simulink model "DCHR_Dispatch_Stateflow_v40"  (R2026a)
settings: Solver=FixedStepDiscrete  StopTime=dchr_stop_v40  FixedStep=dchr_dt_v40
model workspace (MAT data in the model file):
  dchr_E0_v40 = 9
  dchr_c_v40 = [8 0.25 0.25 64]
  dchr_dt_v40 = 1
  dchr_h_v40 = [8 0.45 1.2 8 0.08 0 4 0 0]
  dchr_input_v40 = [0  6  35  75  0  45; 1  0  35  75  5  45]
  dchr_m0_v40 = [1; 0; 0; 0]
  dchr_p_v40 = [1 10 3 4 0.9 0.8 0.1 5 0.2 20 2]
  dchr_stop_v40 = 1
settings Model: Creator=Lysda  LastModifiedBy=Lysda

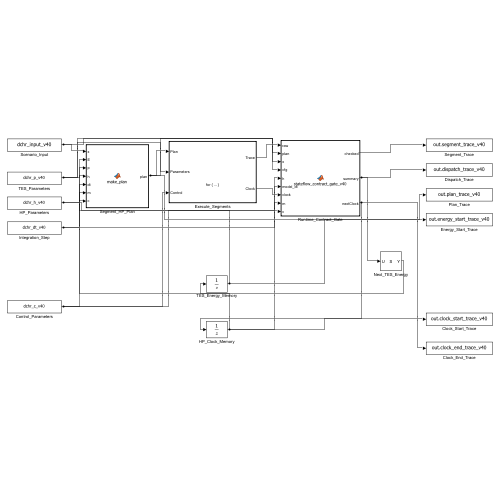
[thumbnail: Simulink's stored preview of the top-level diagram]
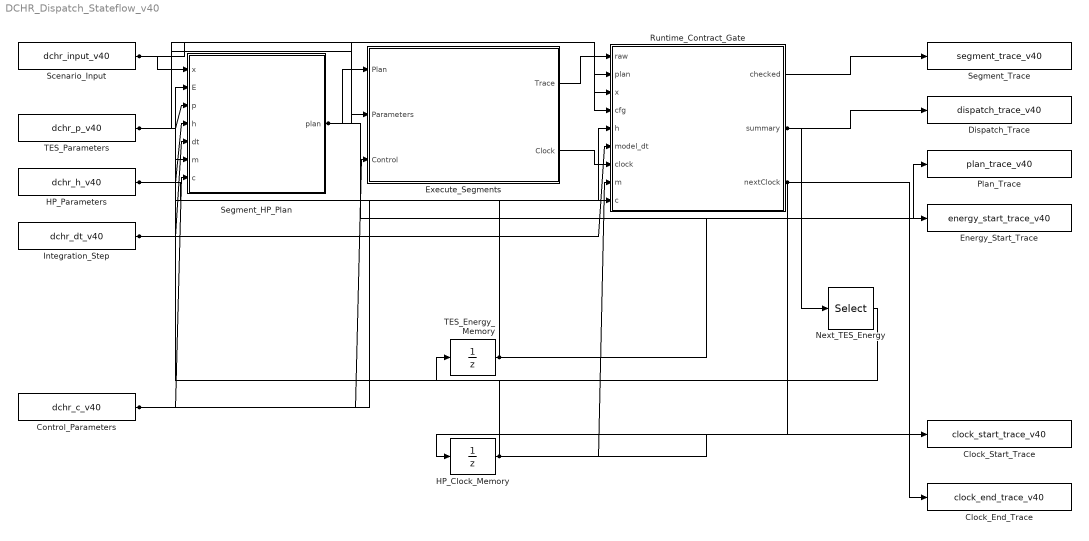
== system DCHR_Dispatch_Stateflow_v40 ==
  Clock_End_Trace : ToWorkspace  VariableName=clock_end_trace_v40  SaveFormat=Timeseries  SampleTime=-1
  Clock_Start_Trace : ToWorkspace  VariableName=clock_start_trace_v40  SaveFormat=Timeseries  SampleTime=-1
  Control_Parameters : Constant  Value=dchr_c_v40
  Dispatch_Trace : ToWorkspace  VariableName=dispatch_trace_v40  SaveFormat=Timeseries  SampleTime=-1
  Energy_Start_Trace : ToWorkspace  VariableName=energy_start_trace_v40  SaveFormat=Timeseries  SampleTime=-1
  Execute_Segments : Subsystem  TreatAsAtomicUnit=on
  HP_Clock_Memory : UnitDelay  InitialCondition=dchr_m0_v40  SampleTime=dchr_dt_v40
  HP_Parameters : Constant  Value=dchr_h_v40
  Integration_Step : Constant  Value=dchr_dt_v40
  Next_TES_Energy : Selector  InputPortWidth=25  IndexOptions=Index vector (dialog)  Indices=8  OutputSizes=1
  Plan_Trace : ToWorkspace  VariableName=plan_trace_v40  SaveFormat=Timeseries  SampleTime=-1
  Runtime_Contract_Gate : MATLAB Function  TreatAsAtomicUnit=on
  Scenario_Input : FromWorkspace  VariableName=dchr_input_v40  SampleTime=dchr_dt_v40  Interpolate=off  OutputAfterFinalValue=Holding final value
  Segment_HP_Plan : MATLAB Function  TreatAsAtomicUnit=on
  Segment_Trace : ToWorkspace  VariableName=segment_trace_v40  SaveFormat=Timeseries  SampleTime=-1
  TES_Energy_Memory : UnitDelay  InitialCondition=dchr_E0_v40  SampleTime=dchr_dt_v40
  TES_Parameters : Constant  Value=dchr_p_v40
  wires:
  Scenario_Input/1 -> Segment_HP_Plan/1(x), Runtime_Contract_Gate/3(x)
  TES_Energy_Memory/1 -> Segment_HP_Plan/2(E), Energy_Start_Trace/1
  TES_Parameters/1 -> Segment_HP_Plan/3(p), Execute_Segments/2(Parameters), Runtime_Contract_Gate/4(cfg)
  HP_Parameters/1 -> Segment_HP_Plan/4(h), Runtime_Contract_Gate/5(h)
  Integration_Step/1 -> Segment_HP_Plan/5(dt), Runtime_Contract_Gate/6(model_dt)
  Segment_HP_Plan/1(plan) -> Execute_Segments/1(Plan), Runtime_Contract_Gate/2(plan), Plan_Trace/1
  Execute_Segments/1(Trace) -> Runtime_Contract_Gate/1(raw)
  Runtime_Contract_Gate/1(checked) -> Segment_Trace/1
  Runtime_Contract_Gate/2(summary) -> Dispatch_Trace/1, Next_TES_Energy/1
  Next_TES_Energy/1 -> TES_Energy_Memory/1
  HP_Clock_Memory/1 -> Segment_HP_Plan/6(m), Runtime_Contract_Gate/8(m), Clock_Start_Trace/1
  Control_Parameters/1 -> Segment_HP_Plan/7(c), Execute_Segments/3(Control), Runtime_Contract_Gate/9(c)
  Execute_Segments/2(Clock) -> Runtime_Contract_Gate/7(clock)
  Runtime_Contract_Gate/3(nextClock) -> HP_Clock_Memory/1, Clock_End_Trace/1

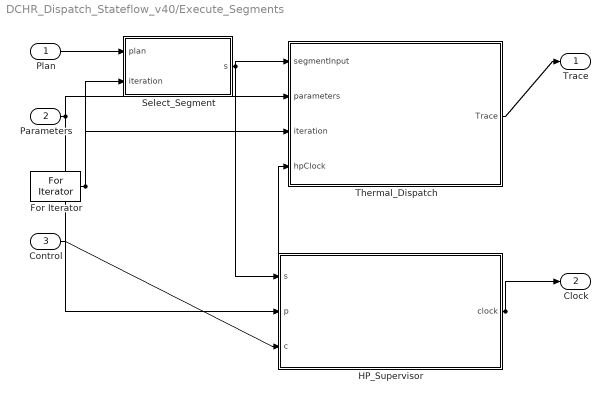
== system DCHR_Dispatch_Stateflow_v40/Execute_Segments ==
  Plan : Inport
  Parameters : Inport  Port=2
  Control : Inport  Port=3
  For Iterator : ForIterator  IterationLimit=64
  HP_Supervisor : Stateflow chart  TreatAsAtomicUnit=on
  Select_Segment : MATLAB Function  TreatAsAtomicUnit=on
  Thermal_Dispatch : Stateflow chart  TreatAsAtomicUnit=on
  Trace : Outport
  Clock : Outport  Port=2
  wires:
  Select_Segment/1(s) -> HP_Supervisor/1(s), Thermal_Dispatch/1(segmentInput)
  Parameters/1 -> HP_Supervisor/2(p), Thermal_Dispatch/2(parameters)
  Control/1 -> HP_Supervisor/3(c)
  HP_Supervisor/1(clock) -> Thermal_Dispatch/4(hpClock), Clock/1
  Plan/1 -> Select_Segment/1(plan)
  For Iterator/1 -> Select_Segment/2(iteration), Thermal_Dispatch/3(iteration)
  Thermal_Dispatch/1(Trace) -> Trace/1

== stateflow chart DCHR_Dispatch_Stateflow_v40/Execute_Segments/HP_Supervisor ==
  settings: description=Persistent HP latch and explicit physical-hour elapsed timer. Safety capacity/input infeasibility overrides ON dwell; OFF dwell remains binding.
  state HP_OFF
    en:
    age=s(16);low=s(19);bound=s(21);
    assert(s(15)==0);
    [age,low,bound]=stateflow_clock_add_v40(age,low,bound,s(1));
    clock=[0;age;low;bound];
    du:
    assert(s(15)==0);
    assert(abs(age-s(16))<=stateflow_time_tolerance_v36([age;s(16)]));
    [age,low,bound]=stateflow_clock_add_v40(age,low,bound,s(1));
    clock=[0;age;low;bound];
  state HP_ON
    en:
    age=s(16);low=s(19);bound=s(21);
    assert(s(15)==1);
    [age,low,bound]=stateflow_clock_add_v40(age,low,bound,s(1));
    clock=[1;age;low;bound];
    du:
    assert(s(15)==1);
    assert(abs(age-s(16))<=stateflow_time_tolerance_v36([age;s(16)]));
    [age,low,bound]=stateflow_clock_add_v40(age,low,bound,s(1));
    clock=[1;age;low;bound];
  (junction 29) -> HP_ON [order 2] : [s(15)==1]
  (default) -> (junction 29)
  (junction 29) -> HP_OFF [order 1] : [s(15)==0]
  HP_ON -> HP_OFF : [s(15)==0 && stateflow_supervisor_guard_v40(0,s,p,c,age,low)]
  HP_OFF -> HP_ON : [s(15)==1 && stateflow_supervisor_guard_v40(1,s,p,c,age,low)]
  data: target function_input; s function_input; p function_input; c function_input; age function_input; low function_input; ok function_output; values function_input; tol function_output; hi function_input; lo function_input; bound function_input; dt function_input; hi function_output; lo function_output; bound function_output; s input double size=[22 1]; p input double size=[1 11]; c input double size=[1 4]; clock output double size=[4 1]; age local double =0; low local double =0; bound local double =0
  function ok=stateflow_supervisor_guard_v40(target,s,p,c,age,low):
    | function ok=stateflow_supervisor_guard_v40(target,s,p,c,age,low)
    | %#codegen
    | % Energy comparisons in MWh; dwell comparisons in physical hours.
    | etol=64*eps(max(1,p(2)));
    | ttol=stateflow_time_tolerance_v36([age;c(2);c(3)]);
    | ok=false;
    | if target==1
    |     ok=s(17)==3 && s(2)<=c(1)+etol && (age-c(3))+low>=0 && s(4)>0 && s(16)==0;
    | else
    |     ok=s(16)==0 && ((s(17)==2 && s(2)>=p(2)-etol && (age-c(2))+low>=0) || ...
    |         (s(17)==1 && s(4)==0));
    | end
    | end
  function tol=stateflow_time_tolerance_v36(values):
    | function tol=stateflow_time_tolerance_v36(values)
    | %#codegen
    | % All inputs and the tolerance are physical HOURS. No energy/power inputs.
    | assert(all(isfinite(values)) && all(values>=0),'Invalid physical-hour scale.');
    | tol=64*eps(max(1,max(abs(values))));
    | % Explicit numerical-resolution contract: never silently relax dwell/clock QA.
    | assert(tol<=1e-8,'Physical-hour resolution exceeds 1e-8 h budget.');
    | end
  function [hi,lo,bound]=stateflow_clock_add_v40(hi,lo,bound,dt):
    | function [hi,lo,bound]=stateflow_clock_add_v40(hi,lo,bound,dt)
    | %#codegen
    | % TwoSum expansion in HOURS. bound encloses discarded low-order roundoff.
    | assert(all(isfinite([hi;lo;bound;dt])) && hi>=0 && bound>=0 && dt>=0,'Invalid compensated clock.');
    | stateflow_time_tolerance_v36([hi;dt]);
    | assert(abs(lo)<=eps(max(1,hi)) && abs(lo)+bound<=1e-8,'Clock cumulative accuracy budget exceeded.');
    | if dt==0,return;end
    | [sumHigh,e]=twosum(hi,dt);
    | [r,discard]=twosum(lo,e);
    | [hi,lo]=twosum(sumHigh,r);
    | candidate=bound+abs(discard);
    | % Conservative upward allowance, including when the addition rounds down.
    | if discard~=0,bound=candidate+eps(candidate);end
    | assert(isfinite(hi) && isfinite(lo) && abs(lo)+bound<=1e-8,'Clock cumulative accuracy budget exceeded.');
    | stateflow_time_tolerance_v36([hi;dt]);
    | end
    | function [sumValue,e]=twosum(a,b)
    | sumValue=a+b;z=sumValue-a;e=(a-(sumValue-z))+(b-z);
    | end

== matlab function DCHR_Dispatch_Stateflow_v40/Runtime_Contract_Gate ==
  data: raw input; checked output; plan input; x input; cfg input; h input; model_dt input; clock input; m input; c input; summary output; nextClock output
function [checked,summary,nextClock]=stateflow_contract_gate_v40(raw,plan,x,cfg,h,model_dt,clock,m,c)
%#codegen
% Per-segment independent ODE/HP/service laws, then integrate powers.
dt=cfg(1);cap=cfg(2);rate=cfg(7);ec=cfg(5);ed=cfg(6);
assert(all(isfinite(cfg)) && dt==model_dt && dt>0,'Invalid model interval.');
assert(all(isfinite(x)) && all(isfinite(h)),'Invalid host inputs.');
energy=zeros(9,1);loss=zeros(3,1);highest=0;
offset=0;previousE=plan(2,1);prevOn=m(1);prevAge=m(2);prevLow=m(3);prevBound=m(4);
for k=1:64
    z=raw((k-1)*28+(1:28));s=plan(:,k);span=z(2);
    finite=z;finite(15)=0;
    assert(all(isfinite(finite)) && all(isfinite(s([1:7 9:14]))),'Nonfinite segment.');
    % Separate dimensional budgets; energy cancellation does not relax clocks.
    tol=1e-10+64*eps(max(1,cap+(h(1)+cfg(11))*dt)); % MWh
    ptol=1e-9+64*eps(max(1,max(abs([x(1);x(4);h(1);cfg(3);cfg(4);cfg(11)])))); % MW
    ktol=1e-9+64*eps(max(1,max(abs([cfg(10);z(22);z(23)])))); % K
    ctol=1e-10+64*eps(max(1,max(abs([h(3);h(4);(x(3)+273.15)/(x(3)-x(2))])))); % dimensionless
    ttol=stateflow_time_tolerance_v36([dt;prevAge;z(27);z(28);c(2);c(3)]); % h
    assert(span>=0 && span==s(1) && z(3)==s(14) && abs(z(4)-s(2))<=tol,'Segment schedule mismatch.');
    assert(z(1)==floor(z(1)) && z(1)>=0 && z(1)<=5,'Undefined segment state.');
    assert(min(z(4:5))>=-tol && max(z(4:5))<=cap+tol,'TES bounds failure.');
    assert(all(z(6:14)>=-ptol) && z(16)>=-ptol && all(z(17:19)>=-tol) && z(20)>=-ptol,'Negative flows/losses.');
    assert(z(7)<=cfg(3)+ptol && z(8)<=cfg(4)+ptol && z(9)<=cfg(11)+ptol && z(7)*z(8)==0,'Instantaneous port limits.');
    if span>0
        P=ec*z(7)-z(8)/ed;r=exp(-rate*span);phi=span;
        if rate>0 && rate*span>0,phi=-expm1(-rate*span)/rate;end
        assert(abs(z(5)-(z(4)*r+P*phi))<=tol,'Segment ODE failure.');
        assert(z(8)==0 || min(z(4:5))>=cfg(8)-tol,'Discharge crosses cutoff.');
        assert(abs(z(17)-(z(4)+P*span-z(5)))<=tol && ...
            abs(z(18)-(1-ec)*z(7)*span)<=tol && abs(z(19)-(1/ed-1)*z(8)*span)<=tol,'Segment losses failure.');
        assert(abs(z(11)-z(12)-z(13))<=ptol && abs(z(11)-z(6)-z(7))<=ptol,'HP first law/allocation failure.');
        assert(abs(x(4)-z(6)-z(8)-z(9)-z(10))<=ptol && ...
            abs(z(20)-z(6)-z(8)-z(9))<=ptol,'Segment service closure.');
        expected=0;
        if z(10)>0,expected=5;elseif z(9)>0,expected=4;elseif z(8)>0,expected=3;
        elseif z(7)>0,expected=2;elseif z(6)>0,expected=1;end
        assert(z(1)==expected,'State does not authorize actual segment flows.');
        assert(abs(x(1)-z(13)-z(16))<=ptol && z(11)<=h(1)+ptol && z(11)<=z(14)+ptol,'Source/request/capacity limit.');
        if z(11)>0
            carnot=(x(3)+273.15)/(x(3)-x(2));
            nominal=h(2)*carnot;if h(6)==1,nominal=h(7)+h(8)*(x(3)-x(2))+h(9)*(x(3)-x(2))^2;end
            expectedCOP=min(h(4),nominal)*(1-h(5)+h(5)*(z(11)/h(1)));
            assert(isfinite(z(15)) && z(15)>=h(3)-ctol && z(15)<=carnot+ctol && z(25)==1 && ...
                abs(z(15)-expectedCOP)<=ctol && abs(z(12)*z(15)-z(11))<=ptol,'Segment COP failure.');
        else,assert(isnan(z(15)) && z(25)==0,'Off HP convention.');end
        highest=max(highest,z(1));
    else
        assert(z(1)==0 && all(z(6:14)==0) && all(z(17:21)==0) && z(5)==z(4),'Zero-span segment has service.');
    end
    assert(abs(z(22)-(cfg(10)+z(4)/cfg(9)))<=ktol && ...
        abs(z(23)-(cfg(10)+z(5)/cfg(9)))<=ktol,'Segment temperature mismatch.');
    residual=z(4)+(z(13)+z(12)+z(9)-z(20))*span-z(5)-sum(z(17:19));
    assert(abs(residual)<=tol && abs(z(21)-residual)<=tol,'Segment system balance failure.');
    assert(z(24)==s(13) && ismember(z(24),[0 1 2 3 4]),'Invalid event kind.');
    assert(abs(z(3)-offset)<=ttol && abs(z(4)-previousE)<=tol,'Ordered event/energy handoff failure.');
    assert(z(26)==s(15) && ismember(z(26),[0 1]) && abs(z(27)-s(16))<=ttol && ...
        abs(z(28)-z(27)-span)<=ttol && abs(z(28)-s(18))<=ttol,'Physical-hour clock failure.');
    if z(26)~=prevOn
        assert(stateflow_supervisor_guard_v40(z(26),s,cfg,c,prevAge,prevLow),'Unauthorized HP latch transition.');
    else
        assert(s(17)==0 && abs(z(27)-prevAge)<=ttol,'Persistent timer continuity failure.');
    end
    if span>0
        assert((z(26)==0 && z(11)==0) || (z(26)==1 && z(11)>0),'HP latch/allocation mismatch.');
    end
    if z(24)==1,assert(abs(z(5)-cap)<=tol,'Capacity event mismatch.');end
    if z(24)==2,assert(abs(z(5)-cfg(8))<=tol,'Cutoff event mismatch.');end
    [wantedAge,wantedLow,wantedBound]=stateflow_clock_add_v40(s(16),s(19),s(21),span);
    assert(s(18)==wantedAge && s(20)==wantedLow && s(22)==wantedBound,'Compensated segment clock mismatch.');
    if z(26)~=prevOn
        assert(s(19)==0 && s(21)==0,'Clock residual/bound reset failure.');
    else
        assert(s(19)==prevLow && s(21)==prevBound,'Persistent residual/bound continuity failure.');
    end
    prevLow=s(20);prevBound=s(22);
    prevOn=z(26);prevAge=z(28);previousE=z(5);offset=offset+span;
    energy=energy+[z(6:14)]*span;loss=loss+z(17:19);
end
first=raw(1:28);last=raw(1765:1792);
tol=1e-10+64*eps(max(1,cap+energy(6)+cfg(11)*dt));
ttol=stateflow_time_tolerance_v36([dt;prevAge;clock(2);c(2);c(3)]);
assert(abs(offset-dt)<=ttol,'Interval partition failure.');
assert(clock(1)==prevOn && abs(clock(2)-prevAge)<=ttol,'Final persistent supervisor clock mismatch.');
assert(clock(3)==prevLow && clock(4)==prevBound,'Supervisor residual/bound mismatch.');
stateflow_clock_add_v40(clock(2),clock(3),clock(4),0);
nextClock=clock;
supplied=(energy(1)+energy(3)+energy(4))/dt;
residual=first(4)+energy(7)+energy(8)+energy(4)-supplied*dt-last(5)-sum(loss);
assert(abs(residual)<=tol,'Integrated first law failure.');
cop=NaN;if energy(7)>0,cop=energy(6)/energy(7);end
summary=[highest;energy(1:5)/dt;first(4)*exp(-rate*dt);last(5);loss;supplied;residual; ...
    first(22);last(23);max(0,first(4)-cfg(8));max(0,last(5)-cfg(8)); ...
    x(4);energy(6:9)/dt;cop;double(energy(6)>0);x(1)-energy(8)/dt];
checked=raw;
end

function ok=stateflow_supervisor_guard_v40(target,s,p,c,age,low)
%#codegen
% Energy comparisons in MWh; dwell comparisons in physical hours.
etol=64*eps(max(1,p(2)));
ttol=stateflow_time_tolerance_v36([age;c(2);c(3)]);
ok=false;
if target==1
    ok=s(17)==3 && s(2)<=c(1)+etol && (age-c(3))+low>=0 && s(4)>0 && s(16)==0;
else
    ok=s(16)==0 && ((s(17)==2 && s(2)>=p(2)-etol && (age-c(2))+low>=0) || ...
        (s(17)==1 && s(4)==0));
end
end

function [hi,lo,bound]=stateflow_clock_add_v40(hi,lo,bound,dt)
%#codegen
% TwoSum expansion in HOURS. bound encloses discarded low-order roundoff.
assert(all(isfinite([hi;lo;bound;dt])) && hi>=0 && bound>=0 && dt>=0,'Invalid compensated clock.');
stateflow_time_tolerance_v36([hi;dt]);
assert(abs(lo)<=eps(max(1,hi)) && abs(lo)+bound<=1e-8,'Clock cumulative accuracy budget exceeded.');
if dt==0,return;end
[sumHigh,e]=twosum(hi,dt);
[r,discard]=twosum(lo,e);
[hi,lo]=twosum(sumHigh,r);
candidate=bound+abs(discard);
% Conservative upward allowance, including when the addition rounds down.
if discard~=0,bound=candidate+eps(candidate);end
assert(isfinite(hi) && isfinite(lo) && abs(lo)+bound<=1e-8,'Clock cumulative accuracy budget exceeded.');
stateflow_time_tolerance_v36([hi;dt]);
end
function [sumValue,e]=twosum(a,b)
sumValue=a+b;z=sumValue-a;e=(a-(sumValue-z))+(b-z);
end

function tol=stateflow_time_tolerance_v36(values)
%#codegen
% All inputs and the tolerance are physical HOURS. No energy/power inputs.
assert(all(isfinite(values)) && all(values>=0),'Invalid physical-hour scale.');
tol=64*eps(max(1,max(abs(values))));
% Explicit numerical-resolution contract: never silently relax dwell/clock QA.
assert(tol<=1e-8,'Physical-hour resolution exceeds 1e-8 h budget.');
end

== matlab function DCHR_Dispatch_Stateflow_v40/Execute_Segments/Select_Segment ==
  data: plan input; s output; iteration input
function s=pick(plan,iteration)
%#codegen
s=plan(:,iteration);
end

== matlab function DCHR_Dispatch_Stateflow_v40/Segment_HP_Plan ==
  data: x input; plan output; E input; p input; h input; dt input; m input; c input
function plan=make_plan(x,E,p,h,dt,m,c)
%#codegen
coder.extrinsic('dchr_segment_plan_v40');
plan=zeros(22,64);
plan=dchr_segment_plan_v40(x,E,p,h,dt,m,c);
end

== stateflow chart DCHR_Dispatch_Stateflow_v40/Execute_Segments/Thermal_Dispatch ==
  settings: description=Release 0.40: bounded physical-hour events, actual persistent HP ON/OFF supervisor and six guarded thermal modes. Normal-mode host HP planner.
  state IDLE
    en,du:
    if iteration==1
    Trace=zeros(1792,1);
    end
    segmentOutput=stateflow_allocate_v40(0,segmentInput,parameters,hpClock);
    Trace=stateflow_collect_v40(Trace,segmentOutput,iteration);
  state HEAT_RECOVERY
    en,du:
    if iteration==1
    Trace=zeros(1792,1);
    end
    segmentOutput=stateflow_allocate_v40(1,segmentInput,parameters,hpClock);
    Trace=stateflow_collect_v40(Trace,segmentOutput,iteration);
  state STORAGE_CHARGE
    en,du:
    if iteration==1
    Trace=zeros(1792,1);
    end
    segmentOutput=stateflow_allocate_v40(2,segmentInput,parameters,hpClock);
    Trace=stateflow_collect_v40(Trace,segmentOutput,iteration);
  state STORAGE_DISCHARGE
    en,du:
    if iteration==1
    Trace=zeros(1792,1);
    end
    segmentOutput=stateflow_allocate_v40(3,segmentInput,parameters,hpClock);
    Trace=stateflow_collect_v40(Trace,segmentOutput,iteration);
  state BACKUP
    en,du:
    if iteration==1
    Trace=zeros(1792,1);
    end
    segmentOutput=stateflow_allocate_v40(4,segmentInput,parameters,hpClock);
    Trace=stateflow_collect_v40(Trace,segmentOutput,iteration);
  state UNMET_DEMAND
    en,du:
    if iteration==1
    Trace=zeros(1792,1);
    end
    segmentOutput=stateflow_allocate_v40(5,segmentInput,parameters,hpClock);
    Trace=stateflow_collect_v40(Trace,segmentOutput,iteration);
  (junction 28) -> STORAGE_CHARGE [order 3] : [stateflow_choose_mode_v40(segmentInput,parameters)==2]
  (junction 28) -> HEAT_RECOVERY [order 2] : [stateflow_choose_mode_v40(segmentInput,parameters)==1]
  (default) -> (junction 28)
  (junction 28) -> IDLE [order 1] : [stateflow_choose_mode_v40(segmentInput,parameters)==0]
  (junction 28) -> UNMET_DEMAND [order 6] : [stateflow_choose_mode_v40(segmentInput,parameters)==5]
  (junction 28) -> STORAGE_DISCHARGE [order 4] : [stateflow_choose_mode_v40(segmentInput,parameters)==3]
  (junction 28) -> BACKUP [order 5] : [stateflow_choose_mode_v40(segmentInput,parameters)==4]
  STORAGE_CHARGE -> STORAGE_DISCHARGE [order 3] : [stateflow_choose_mode_v40(segmentInput,parameters)==3]
  HEAT_RECOVERY -> STORAGE_DISCHARGE [order 3] : [stateflow_choose_mode_v40(segmentInput,parameters)==3]
  STORAGE_CHARGE -> BACKUP [order 4] : [stateflow_choose_mode_v40(segmentInput,parameters)==4]
  UNMET_DEMAND -> IDLE [order 1] : [stateflow_choose_mode_v40(segmentInput,parameters)==0]
  STORAGE_DISCHARGE -> IDLE [order 1] : [stateflow_choose_mode_v40(segmentInput,parameters)==0]
  STORAGE_CHARGE -> IDLE [order 1] : [stateflow_choose_mode_v40(segmentInput,parameters)==0]
  BACKUP -> IDLE [order 1] : [stateflow_choose_mode_v40(segmentInput,parameters)==0]
  HEAT_RECOVERY -> IDLE [order 1] : [stateflow_choose_mode_v40(segmentInput,parameters)==0]
  STORAGE_DISCHARGE -> HEAT_RECOVERY [order 2] : [stateflow_choose_mode_v40(segmentInput,parameters)==1]
  STORAGE_DISCHARGE -> STORAGE_CHARGE [order 3] : [stateflow_choose_mode_v40(segmentInput,parameters)==2]
  BACKUP -> HEAT_RECOVERY [order 2] : [stateflow_choose_mode_v40(segmentInput,parameters)==1]
  UNMET_DEMAND -> HEAT_RECOVERY [order 2] : [stateflow_choose_mode_v40(segmentInput,parameters)==1]
  STORAGE_CHARGE -> HEAT_RECOVERY [order 2] : [stateflow_choose_mode_v40(segmentInput,parameters)==1]
  IDLE -> HEAT_RECOVERY [order 1] : [stateflow_choose_mode_v40(segmentInput,parameters)==1]
  IDLE -> STORAGE_CHARGE [order 2] : [stateflow_choose_mode_v40(segmentInput,parameters)==2]
  BACKUP -> STORAGE_CHARGE [order 3] : [stateflow_choose_mode_v40(segmentInput,parameters)==2]
  UNMET_DEMAND -> STORAGE_CHARGE [order 3] : [stateflow_choose_mode_v40(segmentInput,parameters)==2]
  HEAT_RECOVERY -> STORAGE_CHARGE [order 2] : [stateflow_choose_mode_v40(segmentInput,parameters)==2]
  IDLE -> STORAGE_DISCHARGE [order 3] : [stateflow_choose_mode_v40(segmentInput,parameters)==3]
  HEAT_RECOVERY -> BACKUP [order 4] : [stateflow_choose_mode_v40(segmentInput,parameters)==4]
  STORAGE_CHARGE -> UNMET_DEMAND [order 5] : [stateflow_choose_mode_v40(segmentInput,parameters)==5]
  IDLE -> BACKUP [order 4] : [stateflow_choose_mode_v40(segmentInput,parameters)==4]
  IDLE -> UNMET_DEMAND [order 5] : [stateflow_choose_mode_v40(segmentInput,parameters)==5]
  HEAT_RECOVERY -> UNMET_DEMAND [order 5] : [stateflow_choose_mode_v40(segmentInput,parameters)==5]
  UNMET_DEMAND -> STORAGE_DISCHARGE [order 4] : [stateflow_choose_mode_v40(segmentInput,parameters)==3]
  BACKUP -> STORAGE_DISCHARGE [order 4] : [stateflow_choose_mode_v40(segmentInput,parameters)==3]
  UNMET_DEMAND -> BACKUP [order 5] : [stateflow_choose_mode_v40(segmentInput,parameters)==4]
  STORAGE_DISCHARGE -> BACKUP [order 4] : [stateflow_choose_mode_v40(segmentInput,parameters)==4]
  STORAGE_DISCHARGE -> UNMET_DEMAND [order 5] : [stateflow_choose_mode_v40(segmentInput,parameters)==5]
  BACKUP -> UNMET_DEMAND [order 5] : [stateflow_choose_mode_v40(segmentInput,parameters)==5]
  data: seg function_input; cfg function_input; mode function_output; mode function_input; seg function_input; cfg function_input; clock function_input; z function_output; previous function_input; z function_input; index function_input; packed function_output; segmentInput input double size=[22 1]; parameters input double size=[1 11]; iteration input int32 size=1; hpClock input double size=[4 1]; Trace output double size=[1792 1]; segmentOutput local double size=[28 1]
  function mode=stateflow_choose_mode_v40(seg,cfg):
    | function mode=stateflow_choose_mode_v40(seg,cfg)
    | %#codegen
    | % Guard each positive-duration segment using instantaneous service deficit.
    | direct=min(seg(3),seg(4));remaining=max(0,seg(3)-direct-seg(12));
    | mode=0;
    | if seg(1)==0,return;end
    | if remaining>cfg(11),mode=5;
    | elseif remaining>0,mode=4;
    | elseif seg(12)>0,mode=3;
    | elseif seg(11)>0,mode=2;
    | elseif direct>0,mode=1;
    | end
    | end
  function z=stateflow_allocate_v40(mode,seg,cfg,clock):
    | function z=stateflow_allocate_v40(mode,seg,cfg,clock)
    | %#codegen
    | % Actual Stateflow state authorizes instantaneous TES and finite boiler ports.
    | span=seg(1);A=seg(2);direct=0;qc=0;qd=0;gas=0;unmet=0;
    | if span>0
    |     if mode>=1,direct=min(seg(3),seg(4));end
    |     if mode==2,qc=seg(11);end
    |     if mode>=3,qd=seg(12);end
    |     if mode>=4,gas=min(cfg(11),max(0,seg(3)-direct-qd));end
    |     if mode==5,unmet=max(0,seg(3)-direct-qd-gas);end
    | end
    | P=cfg(5)*qc-qd/cfg(6);rate=cfg(7);x=rate*span;
    | r=exp(-x);f=-expm1(-x);phi=span;beta=0;
    | if rate>0 && x>0
    |     phi=f/rate;
    |     if x<1e-4,beta=span*x*(.5-x*(1/6-x*(1/24-x*(1/120-x/720))));
    |     else,beta=span-phi;end
    | end
    | endpoint=A*r+P*phi;standing=A*f+P*beta;
    | % Roundoff correction only; reject any material bound crossing before clipping.
    | roundoff=64*eps(max(1,cfg(2)));
    | assert(endpoint>=-roundoff && endpoint<=cfg(2)+roundoff,'TES segment crosses physical capacity.');
    | endpoint=min(cfg(2),max(0,endpoint));
    | if qd>0 && seg(13)==2 && abs(endpoint-cfg(8))<=roundoff,endpoint=cfg(8);end
    | lc=(1-cfg(5))*qc*span;ld=(1/cfg(6)-1)*qd*span;
    | supplied=direct+qd+gas;
    | residual=(seg(6)+seg(5)+gas)*span+A-supplied*span-endpoint-standing-lc-ld;
    | z=[mode;span;seg(14);A;endpoint;direct;qc;qd;gas;unmet;seg(4:8);seg(10); ...
    |     standing;lc;ld;supplied;residual;cfg(10)+A/cfg(9);cfg(10)+endpoint/cfg(9);seg(13);seg(9);clock(1);seg(16);clock(2)];
    | end
  function packed=stateflow_collect_v40(previous,z,index):
    | function packed=stateflow_collect_v40(previous,z,index)
    | %#codegen
    | % Bounded event slots; zero-span padding contributes neither energy nor time.
    | assert(index>=1 && index<=64,'Unexpected segment iteration.');
    | packed=previous;
    | if index==1,packed=zeros(1792,1);end
    | packed((double(index)-1)*28+(1:28))=z;
    | end
